simulink model "arducopter"  (R2024b)
settings: Solver=FixedStepAuto  StartTime=0.0  StopTime=simIn.param.timeEnd  FixedStep=simIn.param.dt  RelTol=1e-3
undefined symbols (not defined in the file or in its folder): DiscIntNeverNeededParam, sim, simIn
libraries: simulink x60, slident x4, vrlib x1
(part 9 of 9)

== matlab function arducopter/Attitude Controller/input_euler_angle_roll_pitch_euler_rate_yaw()/thrust_heading_rotation_angles()/thrust_vector_rotation_angles()/MATLAB Function2 ==
  data: thrustErrAngle input; rotVec input; rotVecNorm output
function rotVecNorm = normalizeVec(thrustErrAngle, rotVec)
% Function to normalize the thrust rotation vector. Divides the vector by
% its length or uses up-vector if thrust error angle is zero
rotVecNorm = single(zeros(3,1));
vecLen = single(sqrt(rotVec(1)^2 + rotVec(2)^2 + rotVec(3)^2));

if thrustErrAngle == 0 || vecLen == 0
    rotVecNorm = single([0;0;-1]);
else
    rotVecNorm(1) = rotVec(1) / vecLen;
    rotVecNorm(2) = rotVec(2) / vecLen;
    rotVecNorm(3) = rotVec(3) / vecLen;
end

== matlab function arducopter/Attitude Controller/input_euler_angle_roll_pitch_euler_rate_yaw()/thrust_heading_rotation_angles()/thrust_vector_rotation_angles()/MATLAB Function3 ==
  data: q input; qInv output
function qInv = invertQuat(q)
% Function inverts the rotation of a quaternion.
% Code based on QuaternionT<T>::inverse(void)
% qInv = [q(1);-q(2);-q(3);-q(4)];
qInv = single(zeros(4,1));
qInv(1) = q(1);
qInv(2) = -q(2);
qInv(3) = -q(3);
qInv(4) = -q(4);

== matlab function arducopter/Attitude Controller/input_euler_angle_roll_pitch_euler_rate_yaw()/thrust_heading_rotation_angles()/thrust_vector_rotation_angles()/MATLAB Function4 ==
  data: q input; vecRot output; vec input
function vecRot = rotateByQuat(q, vec)
% Function rotates vector vec by quaternion q. Equivalent to converting the
% input quaternion to a rotation matrix and then multiplying it by the
% vector. This uses the formula
%
%    v2 = v1 + 2 q1 * qv x v1 + 2 qv x qv x v1
%
% where "x" is the cross product (explicitly inlined for performance below), 
% "q1" is the scalar part and "qv" is the vector part of this quaternion
% Code based on Vector3<T> QuaternionT<T>::operator*()

vecRot = vec;

% Compute and cache "qv x v1"
uv = [q(3) * vec(3) - q(4) * vec(2); q(4) * vec(1) - q(2) * vec(3); q(2) * vec(2) - q(3) * vec(1)];

uv(1) = uv(1) + uv(1);
uv(2) = uv(2) + uv(2);
uv(3) = uv(3) + uv(3);
vecRot(1) = vecRot(1) + q(1) * uv(1) + q(3) * uv(3) - q(4) * uv(2);
vecRot(2) = vecRot(2) + q(1) * uv(2) + q(4) * uv(1) - q(2) * uv(3);
vecRot(3) = vecRot(3) + q(1) * uv(3) + q(2) * uv(2) - q(3) * uv(1);

== matlab function arducopter/Attitude Controller/input_euler_angle_roll_pitch_euler_rate_yaw()/thrust_heading_rotation_angles()/thrust_vector_rotation_angles()/MATLAB Function5 ==
  data: axis input; angle input; q output
function q = fromAxisAngle(axis, angle)
% Create a quaternion from its axis-angle representation. The axis-vector
% must be of length 1 and the angle in radians.
% Based on QuaternionT<T>::from_axis_angle()

q = single(zeros(4,1));

if angle == 0
    q(1) = 1;
    q(2) = 0;
    q(3) = 0;
    q(4) = 0;
else
    st2 = sin(0.5*angle);
    q(1) = cos(0.5*angle);
    q(2) = axis(1) * st2;
    q(3) = axis(2) * st2;
    q(4) = axis(3) * st2;
end

== matlab function arducopter/Attitude Controller/input_euler_angle_roll_pitch_euler_rate_yaw()/thrust_heading_rotation_angles()/thrust_vector_rotation_angles()/MATLAB Function6 ==
  data: q input; vec output single
function vec = toAxisAngle(q)
% Converts the quaternion to a rotation vector. The direction represents
% the axis of rotation and the length represents the angle of rotation
% Code based on QuaternionT<T>::to_axis_angle()
l = sqrt(q(2)^2 + q(3)^2 + q(4)^2);

vec = [q(2);q(3);q(4)];

if l ~= 0
    vec = vec ./ l;
    mult = 2 * atan2(l, q(1));
    % The following lines are taken from wrap_pi() in AP_Math.cpp
    mult = mod(mult, 2*pi);
    if mult < 0
        mult = mult + 2*pi;
    end
    if mult > pi
        mult = mult - 2*pi;
    end

    vec = vec .* mult;
end

== matlab function arducopter/Attitude Controller/input_euler_angle_roll_pitch_euler_rate_yaw()/thrust_heading_rotation_angles()/thrust_vector_rotation_angles()/MATLAB Function7 ==
  data: q input; qInv output
function qInv = invertQuat(q)
% Function inverts the rotation of a quaternion.
% Code based on QuaternionT<T>::inverse(void)
% qInv = [q(1);-q(2);-q(3);-q(4)];
qInv = single(zeros(4,1));
qInv(1) = q(1);
qInv(2) = -q(2);
qInv(3) = -q(3);
qInv(4) = -q(4);

== matlab function arducopter/Attitude Controller/input_euler_angle_roll_pitch_euler_rate_yaw()/thrust_heading_rotation_angles()/thrust_vector_rotation_angles()/MATLAB Function8 ==
  data: q input; qInv output
function qInv = invertQuat(q)
% Function inverts the rotation of a quaternion.
% Code based on QuaternionT<T>::inverse(void)
qInv = [q(1);-q(2);-q(3);-q(4)];

== matlab function arducopter/Attitude Controller/input_euler_angle_roll_pitch_euler_rate_yaw()/thrust_heading_rotation_angles()/thrust_vector_rotation_angles()/MATLAB Function9 ==
  data: q1 input; qRes output; q2 input
function qRes = quatMult(q1, q2)
% Quaternion multiplication. Code based on QuaternionT<T>::operator*() in
% quaternion.cpp

qRes = single(zeros(4,1));
qRes(1) = q1(1)*q2(1) - q1(2)*q2(2) - q1(3)*q2(3) - q1(4)*q2(4);
qRes(2) = q1(1)*q2(2) + q1(2)*q2(1) + q1(3)*q2(4) - q1(4)*q2(3);
qRes(3) = q1(1)*q2(3) - q1(2)*q2(4) + q1(3)*q2(1) + q1(4)*q2(2);
qRes(4) = q1(1)*q2(4) + q1(2)*q2(3) - q1(3)*q2(2) + q1(4)*q2(1);

== matlab function arducopter/Throttle/Throttle Calculations/Boost and Premixing/Throttle_In Handling ==
  data: thrTar input; angBst input; thrHover input; thrOut output; angBstEna input; thrAvgMax output single; thrRpyMix input
function [thrOut, thrAvgMax] = fcn(thrTar, angBst, thrHover, angBstEna, thrRpyMix)
% The following lines represent the set_throttle_out() function in
% AC_AttitudeControl_Multi.cpp, that takes the desired throttle from the
% pilot and calculate the boosted and average max throttle.
if(angBstEna)
    % Reference: AC_AttitudeControl_Multi::get_throttle_boosted(throttle_in)
    thrOut = thrTar + angBst;
else
    thrOut = thrTar;
end

%% Determine throttle_avg_max
thr_des_max = max(thrOut, thrTar);

% The following lines are taken from get_throttle_avg_max()
% Limit throttle_max to [0,1]
thr_des_max = min(max( thr_des_max, single(0)), single(1));

% Calculate maximum throttle between input throttle and needed throttle
% considering mix between roll/pitch and hovering
thrAvgMax = max(thr_des_max, thr_des_max * max( single(0), (single(1) - thrRpyMix) ) + thrHover * thrRpyMix);

== matlab function arducopter/Attitude Controller/input_euler_angle_roll_pitch_euler_rate_yaw()/thrust_heading_rotation_angles()/thrust_vector_rotation_angles()/MATLAB Function10 ==
  data: q input; vec output single
function vec = toAxisAngle(q)
% Converts the quaternion to a rotation vector. The direction represents
% the axis of rotation and the length represents the angle of rotation
% Code based on QuaternionT<T>::to_axis_angle()
l = sqrt(q(2)^2 + q(3)^2 + q(4)^2);

vec = [q(2);q(3);q(4)];

if l ~= 0
    vec = vec ./ l;
    mult = 2 * atan2(l, q(1));
    % The following lines are taken from wrap_pi() in AP_Math.cpp
    mult = mod(mult, 2*pi);
    if mult < 0
        mult = mult + 2*pi;
    end
    if mult > pi
        mult = mult - 2*pi;
    end

    vec = vec .* mult;
end

== matlab function arducopter/Attitude Controller/input_euler_angle_roll_pitch_euler_rate_yaw()/thrust_heading_rotation_angles()/thrust_vector_rotation_angles()/MATLAB Function11 ==
  data: q1 input; qRes output; q2 input
function qRes = quatMult(q1, q2)
% Quaternion multiplication. Code based on QuaternionT<T>::operator*() in
% quaternion.cpp

qRes = single(zeros(4,1));
qRes(1) = q1(1)*q2(1) - q1(2)*q2(2) - q1(3)*q2(3) - q1(4)*q2(4);
qRes(2) = q1(1)*q2(2) + q1(2)*q2(1) + q1(3)*q2(4) - q1(4)*q2(3);
qRes(3) = q1(1)*q2(3) - q1(2)*q2(4) + q1(3)*q2(1) + q1(4)*q2(2);
qRes(4) = q1(1)*q2(4) + q1(2)*q2(3) - q1(3)*q2(2) + q1(4)*q2(1);

== matlab function arducopter/Attitude Controller/input_euler_angle_roll_pitch_euler_rate_yaw()/thrust_heading_rotation_angles()/thrust_vector_rotation_angles()/MATLAB Function12 ==
  data: q1 input; qRes output; q2 input
function qRes = quatMult(q1, q2)
% Quaternion multiplication. Code based on QuaternionT<T>::operator*() in
% quaternion.cpp

qRes = single(zeros(4,1));
qRes(1) = q1(1)*q2(1) - q1(2)*q2(2) - q1(3)*q2(3) - q1(4)*q2(4);
qRes(2) = q1(1)*q2(2) + q1(2)*q2(1) + q1(3)*q2(4) - q1(4)*q2(3);
qRes(3) = q1(1)*q2(3) - q1(2)*q2(4) + q1(3)*q2(1) + q1(4)*q2(2);
qRes(4) = q1(1)*q2(4) + q1(2)*q2(3) - q1(3)*q2(2) + q1(4)*q2(1);

== matlab function arducopter/Attitude Controller/input_euler_angle_roll_pitch_euler_rate_yaw()/thrust_heading_rotation_angles()/thrust_vector_rotation_angles()/MATLAB Function13 ==
  data: q input; qInv output
function qInv = invertQuat(q)
% Function inverts the rotation of a quaternion.
% Code based on QuaternionT<T>::inverse(void)
qInv = [q(1);-q(2);-q(3);-q(4)];

== matlab function arducopter/Attitude Controller/input_euler_angle_roll_pitch_euler_rate_yaw()/thrust_heading_rotation_angles()/thrust_vector_rotation_angles()/MATLAB Function14 ==
  data: q input; qInv output
function qInv = invertQuat(q)
% Function inverts the rotation of a quaternion.
% Code based on QuaternionT<T>::inverse(void)
qInv = [q(1);-q(2);-q(3);-q(4)];

== matlab function arducopter/Attitude Controller/input_euler_angle_roll_pitch_euler_rate_yaw()/thrust_heading_rotation_angles()/thrust_vector_rotation_angles()/MATLAB Function15 ==
  data: q1 input; qRes output; q2 input
function qRes = quatMult(q1, q2)
% Quaternion multiplication. Code based on QuaternionT<T>::operator*() in
% quaternion.cpp

qRes = single(zeros(4,1));
qRes(1) = q1(1)*q2(1) - q1(2)*q2(2) - q1(3)*q2(3) - q1(4)*q2(4);
qRes(2) = q1(1)*q2(2) + q1(2)*q2(1) + q1(3)*q2(4) - q1(4)*q2(3);
qRes(3) = q1(1)*q2(3) - q1(2)*q2(4) + q1(3)*q2(1) + q1(4)*q2(2);
qRes(4) = q1(1)*q2(4) + q1(2)*q2(3) - q1(3)*q2(2) + q1(4)*q2(1);

== matlab function arducopter/Attitude Controller/input_euler_angle_roll_pitch_euler_rate_yaw()/thrust_heading_rotation_angles()/thrust_vector_rotation_angles()/MATLAB Function16 ==
  data: q input; vec output
function vec = toAxisAngle(q)
% Converts the quaternion to a rotation vector. The direction represents
% the axis of rotation and the length represents the angle of rotation
% Code based on QuaternionT<T>::to_axis_angle()
l = sqrt(q(2)^2 + q(3)^2 + q(4)^2);

vec = [q(2);q(3);q(4)];

if l ~= 0
    vec = vec ./ l;
    mult = 2 * atan2(l, q(1));
    % The following lines are taken from wrap_pi() in AP_Math.cpp
    mult = mod(mult, 2*pi);
    if mult < 0
        mult = mult + 2*pi;
    end
    if mult > pi
        mult = mult - 2*pi;
    end

    vec = vec .* mult;
end

== matlab function arducopter/Rate Controller/PID Roll Rate/MATLAB Function ==
  data: p_in input; p_out output; d_in input; pd_max input; d_out output; boost input
function [p_out, d_out] = pd_sum_limit(p_in, d_in, pd_max, boost)
% Code is based on AC_PID::update_all() in AC_PID.cpp

% Boost output if required

p_out = p_in * boost;
d_out = d_in * boost;

% Apply PD sum limit if enabled
if (pd_max > 0)
    pd_sum = abs(p_in + d_in);
    if (pd_sum > pd_max)
        PD_scale = pd_max / pd_sum;
        p_out = p_in * PD_scale;
        d_out = d_in * PD_scale;
    end
end

== matlab function arducopter/Position Controller/PID Acceleration z/MATLAB Function ==
  data: p_in input; p_out output; d_in input; pd_max input; d_out output
function [p_out, d_out] = pd_sum_limit(p_in, d_in, pd_max)

p_out = p_in;
d_out = d_in;

if (pd_max > 0)
    pd_sum = abs(p_in + d_in);
    if (pd_sum > pd_max)
        pd_scale = pd_max / pd_sum;
        p_out = p_in * pd_scale;
        d_out = d_in * pd_scale;
    end
end

== matlab function arducopter/MATLAB Function ==
  data: thrSlewRate input; pd_scale output; angle_p_scale output; thrGBoost input
function [pd_scale, angle_p_scale] = update_throttle_gain_boost(thrSlewRate, thrGBoost)
% Code based on AC_AttitudeControl_Multi::update_throttle_gain_boost()

% default angle-p/pd throttle boost threshold
THR_G_BOOST_THRESH = 1; 

if thrSlewRate > THR_G_BOOST_THRESH
    pd_boost = min(max(thrGBoost + 1, 1), 2);
    pd_scale = [pd_boost; pd_boost; 1];

    p_boost = min(max((thrGBoost + 1) * (thrGBoost + 1), 1), 4);
    angle_p_scale = [p_boost; p_boost; 1];

else
    % reset after every loop and not overridden 
    pd_scale = single([1; 1; 1]);
    angle_p_scale = single([1; 1; 1]);
end

== matlab function arducopter/Rate Controller/PID Pitch Rate/MATLAB Function ==
  data: p_in input; p_out output; d_in input; pd_max input; d_out output; boost input
function [p_out, d_out] = pd_sum_limit(p_in, d_in, pd_max, boost)
% Code is based on AC_PID::update_all() in AC_PID.cpp

% Boost output if required

p_out = p_in * boost;
d_out = d_in * boost;

% Apply PD sum limit if enabled
if (pd_max > 0)
    pd_sum = abs(p_in + d_in);
    if (pd_sum > pd_max)
        PD_scale = pd_max / pd_sum;
        p_out = p_in * PD_scale;
        d_out = d_in * PD_scale;
    end
end

== matlab function arducopter/Attitude Controller/input_euler_angle_roll_pitch_euler_rate_yaw()/update_ang_vel_target_from_att_error()/Calc angular velocity target roll/Square Root Controller ==
  data: err input; correction_rate output; p input; second_ord_lim input; dt input
function correction_rate = sqrt_controller(err, p, second_ord_lim, dt)
% The square root controller
% Code is taken from sqrt_controller(...) in AP_Math\control.cpp

if (second_ord_lim < 0 || second_ord_lim == 0)
   correction_rate = err * p;
elseif (p == 0)
    % P term is zero, but second order limit is positive
    if (err > 0)
        correction_rate = sqrt(single(2.0) * second_ord_lim * err);
    elseif (err < 0)
        correction_rate = sqrt(single(2.0) * second_ord_lim * -err);
    else
        correction_rate = single(0.0);
    end
else
    % P term and second order limit are positive, hence have been defined
    linear_dist = second_ord_lim / (p * p);
    % Check if error exceeds linear range of controller gain
    if (err > linear_dist)
        correction_rate = sqrt(single(2.0) * second_ord_lim * ( err - (linear_dist / single(2.0)) ));
    elseif (err < -linear_dist)
        correction_rate = -sqrt(single(2.0) * second_ord_lim * ( -err - (linear_dist / single(2.0)) ));
    else
        % Return linearly amplified correction if error is in linear range
        correction_rate = err * p;
    end
end

% Prevent oscillations by over-shooting the error correction in the last
% time step
if (dt ~= 0)
    correction_rate = max( min(correction_rate, abs(err) / dt), -abs(err) / dt);
end

== matlab function arducopter/Attitude Controller/input_euler_angle_roll_pitch_euler_rate_yaw()/update_ang_vel_target_from_att_error()/Calc angular velocity target pitch/Square Root Controller ==
  data: err input; correction_rate output; p input; second_ord_lim input; dt input
function correction_rate = sqrt_controller(err, p, second_ord_lim, dt)
% The square root controller
% Code is taken from sqrt_controller(...) in AP_Math\control.cpp

if (second_ord_lim < 0 || second_ord_lim == 0)
   correction_rate = err * p;
elseif (p == 0)
    % P term is zero, but second order limit is positive
    if (err > 0)
        correction_rate = sqrt(single(2.0) * second_ord_lim * err);
    elseif (err < 0)
        correction_rate = sqrt(single(2.0) * second_ord_lim * -err);
    else
        correction_rate = single(0.0);
    end
else
    % P term and second order limit are positive, hence have been defined
    linear_dist = second_ord_lim / (p * p);
    % Check if error exceeds linear range of controller gain
    if (err > linear_dist)
        correction_rate = sqrt(single(2.0) * second_ord_lim * ( err - (linear_dist / single(2.0)) ));
    elseif (err < -linear_dist)
        correction_rate = -sqrt(single(2.0) * second_ord_lim * ( -err - (linear_dist / single(2.0)) ));
    else
        % Return linearly amplified correction if error is in linear range
        correction_rate = err * p;
    end
end

% Prevent oscillations by over-shooting the error correction in the last
% time step
if (dt ~= 0)
    correction_rate = max( min(correction_rate, abs(err) / dt), -abs(err) / dt);
end

== matlab function arducopter/Attitude Controller/input_euler_angle_roll_pitch_euler_rate_yaw()/update_ang_vel_target_from_att_error()/Calc angular velocity target yaw/Square Root Controller ==
  data: err input; correction_rate output; p input; second_ord_lim input; dt input
function correction_rate = sqrt_controller(err, p, second_ord_lim, dt)
% The square root controller
% Code is taken from sqrt_controller(...) in AP_Math\control.cpp

if (second_ord_lim < 0 || second_ord_lim == 0)
   correction_rate = err * p;
elseif (p == 0)
    % P term is zero, but second order limit is positive
    if (err > 0)
        correction_rate = sqrt(single(2.0) * second_ord_lim * err);
    elseif (err < 0)
        correction_rate = sqrt(single(2.0) * second_ord_lim * -err);
    else
        correction_rate = single(0.0);
    end
else
    % P term and second order limit are positive, hence have been defined
    linear_dist = second_ord_lim / (p * p);
    % Check if error exceeds linear range of controller gain
    if (err > linear_dist)
        correction_rate = sqrt(single(2.0) * second_ord_lim * ( err - (linear_dist / single(2.0)) ));
    elseif (err < -linear_dist)
        correction_rate = -sqrt(single(2.0) * second_ord_lim * ( -err - (linear_dist / single(2.0)) ));
    else
        % Return linearly amplified correction if error is in linear range
        correction_rate = err * p;
    end
end

% Prevent oscillations by over-shooting the error correction in the last
% time step
if (dt ~= 0)
    correction_rate = max( min(correction_rate, abs(err) / dt), -abs(err) / dt);
end

== matlab function arducopter/Throttle/Throttle Calculations/Throttle-Attitude-Mixing/Update Throttle Mix ==
  data: thrMixDes input; thrMix output; thrMixMin input; thrMixMax input; thrOut input; thrIn input; thrHover input; dt input; thrMixAct data_store_memory
function thrMix = updateThrMix(thrMixDes, thrMixMin, thrMixMax, thrOut, thrIn, thrHover, dt)
% The function represents the update_throttle_rpy_mix() function in
% AC_AttitudeControl_Multi.cpp
% The function slowly moves rpy_mix to rpy_mix_des which represents the
% desired mix between hover and thrust throttle.
global thrMixAct

if thrMixAct < thrMixDes
    thrMix = thrMixAct + min(2 * dt, thrMixDes - thrMixAct);
elseif thrMixAct > thrMixDes
    thrMix = thrMixAct - min(0.5 * dt, thrMixAct - thrMixDes);
    
    % If the mix is still higher than that being used, reset immediately
    thrOut = max(thrOut, thrIn);
    % since thrOut >= thrIn at this point, we dont't need to
    % check thrIn < thrHover
    if thrOut < thrHover
        mixUsed = (thrOut - thrIn) / (thrHover - thrIn);
    else
        mixUsed = thrOut / thrHover;
    end
    
    thrMix = min(thrMix, max(mixUsed, thrMixDes));
else   % Added else statement due to compiler error for uninitialized output
    thrMix = thrMixAct;
end

thrMix = min( max( thrMix, thrMixMin), thrMixMax );

== matlab function arducopter/Attitude Controller/input_euler_angle_roll_pitch_euler_rate_yaw()/MATLAB Function2 ==
  data: angVel input; angVelLimited output; angVelRollMax input; angVelPitchMax input; angVelYawMax input
function angVelLimited = ang_vel_limit(angVel, angVelRollMax, angVelPitchMax, angVelYawMax)
% Limits angular velocity (rad/s) in body frame
% Code based on AC_AttitudeControl::ang_vel_limit()

angVelLimited = angVel;
if angVelRollMax == 0 || angVelPitchMax == 0
    if angVelRollMax ~= 0
        angVelLimited(1) = max(min(angVel(1), angVelRollMax), -angVelRollMax);
    end
    if angVelPitchMax ~= 0
        angVelLimited(2) = max(min(angVel(2), angVelPitchMax), -angVelPitchMax);
    end
else
    thrustVecAngVel = [angVel(1) / angVelRollMax; angVel(2) / angVelPitchMax];
    thrustVecLen = single(sqrt(thrustVecAngVel(1)^2 + thrustVecAngVel(2)^2));
    if thrustVecLen > 1
        angVelLimited(1) = thrustVecAngVel(1) * angVelRollMax / thrustVecLen;
        angVelLimited(2) = thrustVecAngVel(2) * angVelPitchMax / thrustVecLen;
    end
end
if angVelYawMax ~= 0
    angVelLimited(3) = max(min(angVel(3), angVelYawMax), -angVelYawMax);
end

== matlab function arducopter/Attitude Controller/input_euler_angle_roll_pitch_euler_rate_yaw()/MATLAB Function7 ==
  data: q input; qInv output
function qInv = invertQuat(q)
% Function inverts the rotation of a quaternion.
% Code based on QuaternionT<T>::inverse(void)
% qInv = [q(1);-q(2);-q(3);-q(4)];
qInv = single(zeros(4,1));
qInv(1) = q(1);
qInv(2) = -q(2);
qInv(3) = -q(3);
qInv(4) = -q(4);

== matlab function arducopter/Attitude Controller/input_euler_angle_roll_pitch_euler_rate_yaw()/MATLAB Function11 ==
  data: q1 input; qRes output; q2 input
function qRes = quatMult(q1, q2)
% Quaternion multiplication. Code based on QuaternionT<T>::operator*() in
% quaternion.cpp

qRes = single(zeros(4,1));
qRes(1) = q1(1)*q2(1) - q1(2)*q2(2) - q1(3)*q2(3) - q1(4)*q2(4);
qRes(2) = q1(1)*q2(2) + q1(2)*q2(1) + q1(3)*q2(4) - q1(4)*q2(3);
qRes(3) = q1(1)*q2(3) - q1(2)*q2(4) + q1(3)*q2(1) + q1(4)*q2(2);
qRes(4) = q1(1)*q2(4) + q1(2)*q2(3) - q1(3)*q2(2) + q1(4)*q2(1);

== matlab function arducopter/Attitude Controller/input_euler_angle_roll_pitch_euler_rate_yaw()/MATLAB Function4 ==
  data: q input; vecRot output; vec input
function vecRot = rotateByQuat(q, vec)
% Function rotates vector vec by quaternion q. Equivalent to converting the
% input quaternion to a rotation matrix and then multiplying it by the
% vector. This uses the formula
%
%    v2 = v1 + 2 q1 * qv x v1 + 2 qv x qv x v1
%
% where "x" is the cross product (explicitly inlined for performance below), 
% "q1" is the scalar part and "qv" is the vector part of this quaternion
% Code based on Vector3<T> QuaternionT<T>::operator*()

vecRot = vec;

% Compute and cache "qv x v1"
uv = [q(3) * vec(3) - q(4) * vec(2); q(4) * vec(1) - q(2) * vec(3); q(2) * vec(2) - q(3) * vec(1)];

uv(1) = uv(1) + uv(1);
uv(2) = uv(2) + uv(2);
uv(3) = uv(3) + uv(3);
vecRot(1) = vecRot(1) + q(1) * uv(1) + q(3) * uv(3) - q(4) * uv(2);
vecRot(2) = vecRot(2) + q(1) * uv(2) + q(4) * uv(1) - q(2) * uv(3);
vecRot(3) = vecRot(3) + q(1) * uv(3) + q(2) * uv(2) - q(3) * uv(1);

== matlab function arducopter/Attitude Controller/input_euler_angle_roll_pitch_euler_rate_yaw()/Add feedforward to angVelBody/MATLAB Function ==
  data: angVelBodyFeedforward input; angVelBodyNew output; angVelBodyIn input; thrustErrorAngle input; yawRateAct input; maxThrustErrorAngle4YawCorr input; feedforwardScaler output
function [angVelBodyNew, feedforwardScaler] = addFeedforwardToTargetAngVel(angVelBodyFeedforward, angVelBodyIn, thrustErrorAngle, yawRateAct, maxThrustErrorAngle4YawCorr)
% Function smoothly adds feedforward angular velocity and yaw input to
% target angular velocity.
% Code based on AC_AttitudeControl::attitude_controller_run_quat()

angVelBodyNew = angVelBodyIn;

feedforwardScaler = single(1);
if thrustErrorAngle > 2 * maxThrustErrorAngle4YawCorr
    % thrustErrorAngle too large. Set target yaw rate to actual rate. Do not
    % add feedforward.
    angVelBodyNew(3) = yawRateAct;
elseif thrustErrorAngle > maxThrustErrorAngle4YawCorr
    % thrustErrorAngle still large. Add feedforward values smoothly.
    feedforwardScaler = 1 - (thrustErrorAngle - maxThrustErrorAngle4YawCorr) / maxThrustErrorAngle4YawCorr;
    angVelBodyNew(1) = angVelBodyNew(1) + angVelBodyFeedforward(1) * feedforwardScaler;
    angVelBodyNew(2) = angVelBodyNew(2) + angVelBodyFeedforward(2) * feedforwardScaler;
    angVelBodyNew(3) = angVelBodyNew(3) + angVelBodyFeedforward(3);
    angVelBodyNew(3) = yawRateAct * (1 - feedforwardScaler) + angVelBodyNew(3) * feedforwardScaler;
else
    % thrustErrorAngle small enough to add feedforward values to target
    % angular rates of controller without smoothing.
    angVelBodyNew = angVelBodyNew + angVelBodyFeedforward;
end

== matlab function arducopter/Attitude Controller/input_euler_angle_roll_pitch_euler_rate_yaw()/Update attitudeTarget/MATLAB Function ==
  data: q input; qNorm output
function qNorm = normalizeQuat(q)
% Function to normalze a quaternion. Code based on
% QuaternionT<T>::normalize()

quatLen = single(sqrt(q(1)^2 + q(2)^2 + q(3)^2 + q(4)^2));
if quatLen ~= 0
    qNorm = q ./ quatLen;
else
    qNorm = q;
end

== matlab function arducopter/Attitude Controller/input_euler_angle_roll_pitch_euler_rate_yaw()/Update attitudeTarget/Rotate target attitude/MATLAB Function5 ==
  data: vec input; q output
function q = fromAxisAngle(vec)
% Create a quaternion from its axis-angle representation. Just the rotation
% vector is given as input.
% Based on QuaternionT<T>::from_axis_angle(Vector3<T>)

q = zeros(4,1);
angle = single(sqrt(vec(1)^2 + vec(2)^2 + vec(3)^2));

if angle == 0
    q(1) = single(1);
    q(2) = single(0);
    q(3) = single(0);
    q(4) = single(0);
else
    axis = vec ./ angle;
    % The following lines are based on QuaternionT<T>::from_axis_angle(const Vector3<T> &axis, T theta)
    if angle == 0
        q(1) = single(1);
        q(2) = single(0);
        q(3) = single(0);
        q(4) = single(0);
    else
        st2 = single(sin(0.5*angle));
        q(1) = single(cos(0.5*angle));
        q(2) = axis(1) * st2;
        q(3) = axis(2) * st2;
        q(4) = axis(3) * st2;
    end
end

== matlab function arducopter/Attitude Controller/input_euler_angle_roll_pitch_euler_rate_yaw()/Update attitudeTarget/Rotate target attitude/MATLAB Function1 ==
  data: q1 input; qRes output; q2 input
function qRes = quatMult(q1, q2)
% Quaternion multiplication. Code based on QuaternionT<T>::operator*() in
% quaternion.cpp

qRes = single(zeros(4,1));
qRes(1) = q1(1)*q2(1) - q1(2)*q2(2) - q1(3)*q2(3) - q1(4)*q2(4);
qRes(2) = q1(1)*q2(2) + q1(2)*q2(1) + q1(3)*q2(4) - q1(4)*q2(3);
qRes(3) = q1(1)*q2(3) - q1(2)*q2(4) + q1(3)*q2(1) + q1(4)*q2(2);
qRes(4) = q1(1)*q2(4) + q1(2)*q2(3) - q1(3)*q2(2) + q1(4)*q2(1);

== matlab function arducopter/Body Frame Rates -> DCM/MATLAB Function1 ==
  data: rotMat input; roll output; pitch output; yaw output
function [roll, pitch, yaw] = to_euler(rotMat)
% Calculate euler angles from a rotation matrix
% Based on Matrix3<T>::to_euler()
cx = single(1);
pitch = single(0);
roll = single(0);
yaw = single(0);

if rotMat(3,1) >= 1
    cx = 2*single(pi);
end
if rotMat(3,1) <= -1
    cx = -2*single(pi);
else
    cx = rotMat(3,1);
end
pitch = -asin(cx);
roll = atan2(rotMat(3,2), rotMat(3,3));
yaw = atan2(rotMat(2,1), rotMat(1,1));

== matlab function arducopter/Body Frame Rates -> DCM/MATLAB Function2 ==
  data: roll input; rotMat output; pitch input; yaw input
function rotMat = fromEuler(roll, pitch, yaw)
% Computes rotation matrix from euler angle vector
% Based on QuaternionT<T>::from_euler()

rotMat = single(zeros(3,3));
cp = single(cos(pitch));
sp = single(sin(pitch));
sr = single(sin(roll));
cr = single(cos(roll));
sy = single(sin(yaw));
cy = single(cos(yaw));

rotMat(1,1) = cp * cy;
rotMat(1,2) = (sr * sp * cy) - (cr * sy);
rotMat(1,3) = (cr * sp * cy) + (sr * sy);
rotMat(2,1) = cp * sy;
rotMat(2,2) = (sr * sp * sy) + (cr * cy);
rotMat(2,3) = (cr * sp * sy) - (sr * cy);
rotMat(3,1) =  -sp;
rotMat(3,2) = sr * cp;
rotMat(3,3) = cr * cp;

== matlab function arducopter/Body Frame Rates -> DCM/MATLAB Function3 ==
  data: dcm input; quaternion output
function quaternion = from_rotation_matrix(dcm)
% Function to calculate quaternion from a given rotation matrix.
% Implemented based on QuaternionT<T>::from_rotation_matrx()

m00 = dcm(1,1);
m11 = dcm(2,2);
m22 = dcm(3,3);
m10 = dcm(2,1);
m01 = dcm(1,2);
m20 = dcm(3,1);
m02 = dcm(1,3);
m21 = dcm(3,2);
m12 = dcm(2,3);

tr = m00 + m11 + m22;

if tr > 0
    S = sqrt(tr+1) * 2;
    qw = 0.25 * S;
    qx = (m21 - m12) / S;
    qy = (m02 - m20) / S;
    qz = (m10 - m01) / S;
elseif ((m00 > m11) && (m00 > m22))
    S = sqrt(1.0 + m00 - m11 - m22) * 2.0;
    qw = (m21 - m12) / S;
    qx = 0.25 * S;
    qy = (m01 + m10) / S;
    qz = (m02 + m20) / S;
elseif (m11 > m22)
    S = sqrt(1.0 + m11 - m00 - m22) * 2.0;
    qw = (m02 - m20) / S;
    qx = (m01 + m10) / S;
    qy = 0.25 * S;
    qz = (m12 + m21) / S;
else
    S = sqrt(1.0 + m22 - m00 - m11) * 2.0;
    qw = (m10 - m01) / S;
    qx = (m02 + m20) / S;
    qy = (m12 + m21) / S;
    qz = 0.25 * S;
end

quaternion = [qw;qx;qy;qz];

== matlab function arducopter/radioIn to controlIn/MATLAB Function ==
  data: rcIn input; angleIn output; deadZone input; radioMin input; radioMax input; trim input; reversed input; highIn input
function angleIn = pwm_to_angle_dz(rcIn, deadZone, radioMin, radioMax, trim, reversed, highIn)
% Computes a angle in centidegree value from the current radio_in value
% using the specified dead_zone and trim
% Code based on RC_Channel::pwm_to_angle_dz() and RC_Channel::pwm_to_angle_dz_trim()

radioTrimHigh = trim + deadZone;
radioTrimLow = trim - deadZone;

if reversed
    reverseMul = -1;
else
    reverseMul = 1;
end

% Dont allow out of range values
rcIn = max(min(rcIn, radioMax), radioMin);

if rcIn > radioTrimHigh && radioMax ~= radioTrimHigh
    angleIn = reverseMul * highIn * (rcIn - radioTrimHigh) / (radioMax  - radioTrimHigh);
elseif rcIn < radioTrimLow && radioTrimLow ~= radioMin
    angleIn = reverseMul * highIn * (rcIn - radioTrimLow) / (radioTrimLow - radioMin);
else
    angleIn = single(0);
end

== matlab function arducopter/radioIn to controlIn/MATLAB Function1 ==
  data: radioIn input; out output; deadZone input; radioTrim input; radioMin input; radioMax input; reversed input
function out = norm_input_dz(radioIn, deadZone, radioTrim, radioMin, radioMax, reversed)
% Code based on RC_Channel::norm_input_dz()
dzMin = radioTrim - deadZone;
dzMax = radioTrim + deadZone;

if reversed
    revMult = -1;
else
    revMult = 1;
end

if radioIn < dzMin && dzMin > radioMin
    out = revMult * (radioIn - dzMin) / (dzMin - radioMin);
elseif radioIn > dzMax && radioMax > dzMax
    out = revMult * (radioIn - dzMax) / (radioMax - dzMax);
else
    out = single(0);
end

out = min(max(out, single(-1)), single(1));

== matlab function arducopter/Rate Controller/PID Pitch Rate/Slew Limiter/Calculate Dmod ==
  data: slew_rate input; Dmod output single; sr_max input; sr_tau input; dt input; time input; pos_event_idx data_store_memory; pos_event_stored data_store_memory; pos_event_ms data_store_memory; neg_event_idx data_store_memory; neg_event_stored data_store_memory; neg_event_ms data_store_memory; modifier_slew_rate data_store_memory; output_slew_rate data_store_memory; max_neg_slew_event_ms data_store_memory; max_pos_slew_event_ms data_store_memory; max_neg_slew_rate data_store_memory; max_pos_slew_rate data_store_memory
function Dmod   = fcn(slew_rate, sr_max, sr_tau, dt, time)
% Code is based on SlewLimiter::modifier() in SlewLimiter.cpp. 

% Define global variables, so that quanitities do not have to be fed back
% to the function
global pos_event_stored;
global pos_event_idx;
global pos_event_ms;
global max_pos_slew_rate;
global max_pos_slew_event_ms;
global neg_event_stored;
global neg_event_idx;
global neg_event_ms;
global max_neg_slew_rate;
global max_neg_slew_event_ms;
global modifier_slew_rate;
global output_slew_rate;

% Definition of constants as done in SlewLimiter.h
SLEWLIMITER_N_EVENTS = uint32(3); % Number of positive and negative consecutive slew rate exceedance events recorded. Set to 3 because of 1-based indexing.
WINDOW_MS = uint32(300); % Time in ms required for half a cycle of the slowest oscillation frequency expected
MODIFIER_GAIN = 1.5; % Ratio of modifier reduction to slew rate exceedance

if (dt < 0)
    Dmod = single(1.0);
    return;
end

now_ms = uint32(time);
decay_alpha = min(dt, sr_tau) / sr_tau;

% Apply a filter to decay maximum seen slew rate once the value had left the window period
attack_alpha = min(2.0 * decay_alpha, 1.0);

%% Calculate maximum slew rate
% Save new maximum slew rates, if oldest maximum is exceeded
% OR decay the peak slew rates (pos. and neg.) if they are outside the
% observed time window
% Never drop PID gains below 10% of configured value
if (slew_rate > max_pos_slew_rate)
    max_pos_slew_rate(:) = slew_rate;
    max_pos_slew_event_ms = now_ms;
elseif (now_ms - max_pos_slew_event_ms > WINDOW_MS)
    max_pos_slew_rate = max_pos_slew_rate * (1.0 - decay_alpha);
end

if (-slew_rate > max_neg_slew_rate)
    max_neg_slew_rate(:) = -slew_rate;
    max_neg_slew_event_ms = now_ms;
elseif (now_ms - max_neg_slew_event_ms > WINDOW_MS)
    max_neg_slew_rate = max_neg_slew_rate * (1.0 - decay_alpha);
end

% Calculate the averaged maximum slew rate
raw_slew_rate = 0.5 * (max_pos_slew_rate + max_neg_slew_rate);
% Calculation of output slew rate
output_slew_rate = output_slew_rate + (raw_slew_rate - output_slew_rate) * attack_alpha;
output_slew_rate = min(raw_slew_rate, output_slew_rate);

% Check if slew limiter is activated
if(sr_max <= 0)
   Dmod = single(1.0);
   return;
end

% Constrain slew rate used for calculation
limited_raw_slew_rate = 0.5 * (min(max_pos_slew_rate, 10 * sr_max) + min(max_neg_slew_rate, 10 * sr_max));


%% Save exceedance events in event time vector
% Store a series of positive slew rate exceedance events
if (~pos_event_stored && slew_rate > sr_max)
    if (pos_event_idx >= SLEWLIMITER_N_EVENTS)
        pos_event_idx(:) = 1;
    end
    pos_event_ms(pos_event_idx) = now_ms;
    pos_event_idx(:) = pos_event_idx + 1;
    pos_event_stored = true;
    neg_event_stored = false;
end

% Store a series of negative slew rate exceedance events
if (~neg_event_stored && -slew_rate > sr_max)
    if (neg_event_idx >= SLEWLIMITER_N_EVENTS)
        neg_event_idx(:) = 1;
    end
    neg_event_ms(neg_event_idx) = now_ms;
    neg_event_idx(:) = neg_event_idx + 1;
    pos_event_stored = false;
    neg_event_stored = true;
end

% Find oldest event time
oldest_ms = now_ms;
for i=1:SLEWLIMITER_N_EVENTS-1
   oldest_ms = min(oldest_ms, pos_event_ms(i));
   oldest_ms = min(oldest_ms, neg_event_ms(i));
end

% When the oldest exceedance event falls outside of the window required for
% the number of exceedance events, apply a further reduction to the maximum
% slew rate. This prevents unwanted gain reductions caused by spikes in the
% demanded angular rates due to changed control modes or similar causes.
modifier_input = limited_raw_slew_rate;
if(now_ms - oldest_ms > SLEWLIMITER_N_EVENTS * WINDOW_MS) % no incrementation of SLEWLIMITER_N_EVENTS because of 1 based indexing
   oldest_time_from_window = single(0.001) * single(now_ms - oldest_ms - SLEWLIMITER_N_EVENTS * WINDOW_MS); 
   modifier_input = modifier_input * single(exp(-oldest_time_from_window / sr_tau));
end

%% Calculation of modifier slew rate

modifier_slew_rate = modifier_slew_rate + (modifier_input - modifier_slew_rate) * attack_alpha;
modifier_slew_rate = min(modifier_slew_rate, modifier_input);

% Calculate modifier. Only has an impact if sr_max is exceeded by averaged
% slew rate.
if(modifier_slew_rate > sr_max)
    Dmod(:) = sr_max / (sr_max + MODIFIER_GAIN * (modifier_slew_rate - sr_max));
else
    Dmod(:) = 1.0;
end

== matlab function arducopter/Throttle/Throttle Calculations/Lowpass Filter/Lowpass Filter with reset ==
  data: thr_in input; out output single; cutoff_freq input; dt input; lastThr input; lastSlew input; slewrate output
function [out, slewrate]  = update_throttle_filter(thr_in, cutoff_freq, dt , lastThr, lastSlew)

persistent buffer idx
% filter size of ring buffer for derivative throttle filter, version 4.6.2 see AP_Motors_Class.h line 329
FILTER_SIZE = 7;
% AP_Motors_Class.cpp line 22
SLEW_FILTER_CUTOFF = 50;

%% The code is based on the apply(sample, dt) function in LowPassFilter.cpp.

% Check if filter is supposed to be filtering
if (cutoff_freq <=0 || dt < 0)
    alpha = single(1);
elseif dt == 0
    alpha = single(0);
else
    % Calculate time constant and alpha value
    T = 1 / (2 * pi * cutoff_freq);
    alpha = dt / (dt + T);
end
% Output calculation
out = lastThr + (thr_in - lastThr) * alpha;

%% Code is based on AP_MotorsMulticopter::update_throttle_filter(), in AP_MotorsMulticopter.cpp.
% If the output surpases the limits [0,1], the filter is reset (according
% to the reset() function in LowPassFilter.cpp.)
if (out < single(0.0))
   out = single(0.0); 

elseif (out > 1.0)
    out = single(1.0);
end

if isempty(buffer)
        buffer = zeros(1,FILTER_SIZE);
        idx = 0;
end
% Update throttleSlewRate filter
if out ~= lastThr
    idx = mod(idx, FILTER_SIZE) + 1;
    buffer(idx) = out;
end


% Calculate slope normalized to seconds
% See DerivativeFilter<T,FILTER_SIZE>::slope(void)
% nested help function from DerivativeFilter<T,FILTER_SIZE>::slope(void)
    function val = f(i)
            id = mod(idx + i - 1, FILTER_SIZE) + 1;
            val = buffer(id);
    end

slope = 2 * 5 * (f(1) - f(-1)) / (2 * dt) ...
    + 4 * 1 * (f(2) - f(-2)) / (4 * dt) ... 
    + 6 * 1 * (f(3) - f(-3)) / (6 * dt);
slope = slope / 32;

if (isnan(slope) || isinf(slope))
    slope = single(0);
end

rate = abs(slope);

% Apply rate to throttle slew filter
% Check if filter is supposed to be filtering
if (SLEW_FILTER_CUTOFF <=0 || dt < 0)
    alpha = single(1);
elseif dt == 0
    alpha = single(0);
else
    % Calculate time constant and alpha value
    T = 1 / (2 * pi * SLEW_FILTER_CUTOFF);
    alpha = dt / (dt + T);
end
% Output calculation
slewrate = lastSlew + (rate - lastSlew) * alpha;
end

== matlab function arducopter/radioIn to controlIn/MATLAB Function3 ==
  data: rcIn input; angleIn output; deadZone input; radioMin input; radioMax input; trim input; reversed input; highIn input
function angleIn = pwm_to_angle_dz(rcIn, deadZone, radioMin, radioMax, trim, reversed, highIn)
% Computes a angle in centidegree value from the current radio_in value
% using the specified dead_zone and trim
% Code based on RC_Channel::pwm_to_angle_dz() and RC_Channel::pwm_to_angle_dz_trim()

radioTrimHigh = trim + deadZone;
radioTrimLow = trim - deadZone;

if reversed
    reverseMul = -1;
else
    reverseMul = 1;
end

% Dont allow out of range values
rcIn = max(min(rcIn, radioMax), radioMin);

if rcIn > radioTrimHigh && radioMax ~= radioTrimHigh
    angleIn = reverseMul * highIn * (rcIn - radioTrimHigh) / (radioMax  - radioTrimHigh);
elseif rcIn < radioTrimLow && radioTrimLow ~= radioMin
    angleIn = reverseMul * highIn * (rcIn - radioTrimLow) / (radioTrimLow - radioMin);
else
    angleIn = single(0);
end

== matlab function arducopter/Rate Controller/PID Pitch Rate/Slew Limiter/Lowpass Filter ==
  data: in input; out output single; alpha input; out_last input
function out  = apply(in, alpha, out_last)
% The code is based on the apply(sample, cutoff_freq, dt) function in
% LowPassFilter.cpp

% Output calculation
out = out_last + (in - out_last) * alpha;

== matlab function arducopter/Attitude Controller/input_euler_angle_roll_pitch_euler_rate_yaw()/reset yaw targets/MATLAB Function5 ==
  data: vec input; q output
function q = fromAxisAngle(vec)
% Create a quaternion from its axis-angle representation. Just the rotation
% vector is given as input.
% Based on QuaternionT<T>::from_axis_angle(Vector3<T>)

q = zeros(4,1);
angle = single(sqrt(vec(1)^2 + vec(2)^2 + vec(3)^2));

if angle == 0
    q(1) = single(1);
    q(2) = single(0);
    q(3) = single(0);
    q(4) = single(0);
else
    axis = vec ./ angle;
    % The following lines are based on QuaternionT<T>::from_axis_angle(const Vector3<T> &axis, T theta)
    if angle == 0
        q(1) = single(1);
        q(2) = single(0);
        q(3) = single(0);
        q(4) = single(0);
    else
        st2 = single(sin(0.5*angle));
        q(1) = single(cos(0.5*angle));
        q(2) = axis(1) * st2;
        q(3) = axis(2) * st2;
        q(4) = axis(3) * st2;
    end
end

== matlab function arducopter/radioIn to controlIn/MATLAB Function2 ==
  data: rcIn input; ctrlIn output; deadZone input; radioMin input; radioMax input; reversed input; highIn input
function ctrlIn = pwm_to_range_dz(rcIn, deadZone, radioMin, radioMax, reversed, highIn)
% Converts a pwm value to a value in the configured range
% Code based on RC_Channel::pwm_to_range_dz()

rcIn = max(min(rcIn, radioMax), radioMin);

if reversed
    rcIn = radioMax - (rcIn - radioMin);
end

radioTrimLow = radioMin + deadZone;

if rcIn > radioTrimLow
    ctrlIn = highIn * (rcIn - radioTrimLow) / (radioMax - radioTrimLow);
else
    ctrlIn = single(0);
end

== matlab function arducopter/Position Controller/calc des climb rate/MATLAB Function ==
  data: ctrlIn input; climbRateDes output; deadZoneThr input; deadZoneRC input; radioMin input; radioMax input; reversed input; highIn input; maxSpeedDn input; maxSpeedUp input
function climbRateDes = get_pilot_desired_climb_rate(ctrlIn, deadZoneThr, deadZoneRC, radioMin, radioMax, reversed, highIn, maxSpeedDn, maxSpeedUp)
% Calculation of the desired climb rate based on the pilot's throttle input
% Based on Copter::get_pilot_desired_climb_rate()

% Ensure a reasonable throttle value
ctrlIn = min(max(ctrlIn, 0), 1000);

% Ensure a reasonable deadzone
thrDz = min(max(deadZoneThr, 0), 400);

% Calculation of mid_stick based on Copter::get_throttle_mid()
rIn = (radioMin + radioMax) / 2;
if reversed
    rIn = radioMax - (rIn - radioMin);
end
radioTrimLow = radioMin + deadZoneRC;
midStick = highIn * (rIn - radioTrimLow) / (radioMax - radioTrimLow);

deadbandTop = midStick + thrDz;
deadbandBottom = midStick - thrDz;

% Check throttle is above, below or in the deadband
if ctrlIn < deadbandBottom
    % Below deadband
    % Get maximum down speed that can be demanded by pilot. If zero, the
    % maximum up speed is used according to get_pilot_speed_dn()
    if maxSpeedDn == 0
        maxSpeedDn = abs(maxSpeedUp);
    end
    climbRateDes = maxSpeedDn * (ctrlIn - deadbandBottom) / deadbandBottom;
elseif ctrlIn > deadbandTop
    % Above deadband
    climbRateDes = maxSpeedUp * (ctrlIn - deadbandTop) / (1000 - deadbandTop);
else
    % In the deadband
    climbRateDes = single(0); 
end
